simulink model "FOCwithLOAD"  (R2024b)
settings: Solver=FixedStepDiscrete  StartTime=0.0  StopTime=inf  RelTol=1e-3
PreLoadFcn:
  | % 自动加载同目录下的 linear_data.m，确保换机/首次打开可直接更新与编译
  | if ~evalin('base', 'exist(''Ts'',''var'') && exist(''pmsm'',''var'') && exist(''SMRC_I_Vsat_thresh'',''var'')')
  |     mdlDir_ = '';
  |     if bdIsLoaded('FOCwithLOAD'), mdlDir_ = fileparts(get_param('FOCwithLOAD', 'FileName')); end
  |     if isempty(mdlDir_), mdlDir_ = fileparts(which('FOCwithLOAD')); end
  |     if isempty(mdlDir_), mdlDir_ = pwd; end
  |     dataFile_ = fullfile(mdlDir_, 'linear_data.m');
  |     if isfile(dataFile_)
  |         assignin('base', 'linearDataFileTmp_', dataFile_);
  |         evalin('base', 'run(linearDataFileTmp_); clear linearDataFileTmp_');
  |     end
  |     clear mdlDir_ dataFile_
  | end
InitFcn:
  | % 自动加载同目录下的 linear_data.m，确保换机/首次打开可直接更新与编译
  | if ~evalin('base', 'exist(''Ts'',''var'') && exist(''pmsm'',''var'') && exist(''SMRC_I_Vsat_thresh'',''var'')')
  |     mdlDir_ = '';
  |     if bdIsLoaded('FOCwithLOAD'), mdlDir_ = fileparts(get_param('FOCwithLOAD', 'FileName')); end
  |     if isempty(mdlDir_), mdlDir_ = fileparts(which('FOCwithLOAD')); end
  |     if isempty(mdlDir_), mdlDir_ = pwd; end
  |     dataFile_ = fullfile(mdlDir_, 'linear_data.m');
  |     if isfile(dataFile_)
  |         assignin('base', 'linearDataFileTmp_', dataFile_);
  |         evalin('base', 'run(linearDataFileTmp_); clear linearDataFileTmp_');
  |     end
  |     clear mdlDir_ dataFile_
  | end
values from neighbouring files (symbols this model uses):
  a_hat = Kt_eff / (pmsm.J * omega_pu_base)    [linear_data.m]
  ADRC_B0 = 6055    [linear_data.m]
  ADRC_Wc = 3.2e-3    (= 0.0032)    [linear_data.m]
  ADRC_Wo = 30    [linear_data.m]
  alpha_ppc = exp(-lambda_ppc*Ts_speed)    [linear_data.m]
  b_hat = pmsm.B/pmsm.J    [linear_data.m]
  beta1 = single(2.0 * w_o)    [linear_data.m]
  beta2_sat_scale = 0.2    [linear_data.m]
  dataType = 'single'    [linear_data.m]
  gamma_reset = 0.9    [linear_data.m]
  inv_a_hat = 1/double(a_hat)    [linear_data.m]
  k_xi = 55    [linear_data.m]
  Kff = 0.98931745    [linear_data.m]
  lambda_ppc = 45    [linear_data.m]
  P_inf_const = 0.004    [linear_data.m]
  PI_params = mcb_SetControllerParameters(pmsm,inverter,PU_System,T_pwm,Ts,Ts_speed)    [linear_data.m]
  pmsm2 = pmsm    [linear_data.m]
  s_limit_sat = 0.9    [linear_data.m]
  speedRPM2mmps = pmlsm.mmps_per_rpm    [linear_data.m]
  target = mcb_SetProcessorDetails('F28379D',PWM_frequency)    [linear_data.m]
  Ts = T_pwm    (= 5e-05)    [linear_data.m]
  Ts_motor = T_pwm/2    (= 2.5e-05)    [linear_data.m]
  Ts_speed = 1*Ts    (= 5e-05)    [linear_data.m]
  w_o = single(200.0)    [linear_data.m]
  z2_limit = single(100.0)    [linear_data.m]
undefined symbols (not defined in the file or in its folder): DiscIntNeverNeededParam, Down, GPTRIP1SEL, GPTRIP2SEL, innerPI, inverter, inverter2, outerPI, pmlsm, pmsm, Tctr, TZ1, TZ2, Up
libraries: c2802xlib x13, simulink x10, c2837xDlib x6, c280xlib x6, slpidlib x5, svdschedulerlib x4, mcbcontrolslib x4, mcbpositiondecoderlib x2, mcbpmsmnonlinearlib x2, autolibpmsmexterior x2, mcbplantlib x2, svdutilitieslib x1
(part 2 of 5)

== system FOCwithLOAD/Motor2 Torque control/Control_System ==
  speed_RPM : Inport
  Iabc_meas_Real : Inport  Port=2
  Pos_PU : Inport  Port=3
  EnClosedLoop : Inport  Port=4
  Idq_ref_Real : Inport  Port=5
  AlignMode2Read : DataStoreRead  DataStoreName=AlignMode2  IndexOptions=Index vector (dialog)  Indices=1  OutputSizes=1
  AlignTheta2Read : DataStoreRead  DataStoreName=AlignTheta2  IndexOptions=Index vector (dialog)  Indices=1  OutputSizes=1
  Closed Loop Control1 : Subsystem  TreatAsAtomicUnit=on
  Switch : Switch  Criteria=u2 > Threshold  Threshold=0.5  SaturateOnIntegerOverflow=off  InputSameDT=off
  ThetaSw : Switch  Criteria=u2 > Threshold  Threshold=0.5  SaturateOnIntegerOverflow=off  InputSameDT=off
  ZeroOL : Constant  Value=0  OutDataTypeStr=single
  Duty_ABC : Outport  VectorParamsAs1DForOutWhenUnconnected=off
  VIdq_debug : Outport  Port=2  VectorParamsAs1DForOutWhenUnconnected=off
  wires:
  speed_RPM/1 -> Closed Loop Control1/3(Speed(RPM))
  AlignMode2Read/1 -> ThetaSw/2
  Pos_PU/1 -> ThetaSw/3
  Closed Loop Control1/2(VIdq_debug) -> VIdq_debug/1
  EnClosedLoop/1 -> Closed Loop Control1/Enable, Switch/2
  Idq_ref_Real/1 -> Closed Loop Control1/4(IdqRef)
  Iabc_meas_Real/1 -> Closed Loop Control1/1(Iabc)
  ThetaSw/1 -> Closed Loop Control1/2(Thetae_Sensor(0-1))
  Closed Loop Control1/1(Duty) -> Switch/1
  ZeroOL/1 -> Switch/3
  Switch/1 -> Duty_ABC/1
  AlignTheta2Read/1 -> ThetaSw/1

== system FOCwithLOAD/Motor2 Torque control/HW_Inputs ==
  Sim : Inport
  Sensor Driver Blocks (codegen) : Subsystem  VariantControl=(codegen)
  Sensor Driver Blocks (sim) : Subsystem  VariantControl=(sim)
  Out : Outport

== system FOCwithLOAD/Motor2 Torque control/Input Scaling ==
  note: Current Measurements
  note: Position & Speed Measurements
  note: QEP
  Ia_ADC : Inport
  Ib_ADC : Inport  Port=2
  Ic_ADC : Inport  Port=3
  QEP_Position_Count : Inport  Port=4
  QEP_Index_Latch : Inport  Port=5
  " Calculate Position and Speed" : Subsystem
  Calculate Phase Currents : Subsystem
  UnusedOffset : Constant  Value=0
  speed_RPM : Outport
  Iabc_meas_Real : Outport  Port=2
  Pos_PU : Outport  Port=3
  Motor2IndexFound : Outport  Port=4
  wires:
  Calculate Phase Currents/1(Iabc_meas_Real) -> Iabc_meas_Real/1  "Iabc_fb_Real"
  Ia_ADC/1 -> Calculate Phase Currents/1(Ia_ADC)
  Ib_ADC/1 -> Calculate Phase Currents/2(Ib_ADC)
  Ic_ADC/1 -> Calculate Phase Currents/3(Ic_ADC)
  QEP_Position_Count/1 -> " Calculate Position and Speed"/1(QEP_Position_Count)
  QEP_Index_Latch/1 -> " Calculate Position and Speed"/2(QEP_Index_Latch)
  UnusedOffset/1 -> " Calculate Position and Speed"/3(Offset)
  " Calculate Position and Speed"/1(Theta_e) -> Pos_PU/1
  " Calculate Position and Speed"/2(speed) -> speed_RPM/1
  " Calculate Position and Speed"/3(IndexFound) -> Motor2IndexFound/1

== system FOCwithLOAD/Motor2 Torque control/Inverter ==
  Inverter Signals : Inport
  Code Generation : Subsystem  VariantControl=(codegen)
  Simulation : Subsystem  VariantControl=(sim)
  DutyCycles : Outport  VectorParamsAs1DForOutWhenUnconnected=off

== system FOCwithLOAD/Motor2 Torque control/Output Scaling ==
  DutyABC : Inport
  Data Store Read : DataStoreRead  DataStoreName=EnMtr2Ctrl  IndexOptions=Index vector (dialog)  Indices=1  OutputSizes=1
  Data Type Conversion : DataTypeConversion  OutDataTypeStr=dataType  SaturateOnIntegerOverflow=off  RndMeth=Floor
  PWM_Duty_Cycles : Outport
  PWM_Enable : Outport  Port=2
  wires:
  Data Store Read/1 -> Data Type Conversion/1  "PWM_En"
  Data Type Conversion/1 -> PWM_Enable/1
  DutyABC/1 -> PWM_Duty_Cycles/1

== system FOCwithLOAD/Motor2 Torque control/align ==
  Iq_ref_real : Inport
  AlignMode2Read : DataStoreRead  DataStoreName=AlignMode2  IndexOptions=Index vector (dialog)  Indices=1  OutputSizes=1
  Constant : Constant  Value=0  OutDataTypeStr=single
  IdAlign2 : Constant  Value=1.5  OutDataTypeStr=single
  IdSw2 : Switch  Threshold=0.5  SaturateOnIntegerOverflow=off  InputSameDT=off
  IqSw2 : Switch  Threshold=0.5  SaturateOnIntegerOverflow=off  InputSameDT=off
  Mux1 : Mux  Inputs=2
  Out1 : Outport
  wires:
  Mux1/1 -> Out1/1
  IqSw2/1 -> Mux1/2
  IdSw2/1 -> Mux1/1
  Constant/1 -> IqSw2/1, IdSw2/3
  IdAlign2/1 -> IdSw2/1
  AlignMode2Read/1 -> IdSw2/2, IqSw2/2
  Iq_ref_real/1 -> IqSw2/3

== system FOCwithLOAD/Serial Receive/Parse SCI Rx ==
  Rx : Inport
  CalModeDTC : DataTypeConversion  OutDataTypeStr=uint8  RndMeth=Floor
  CalModeWrite : DataStoreWrite  DataStoreName=CalMode  IndexOptions=Index vector (dialog)  Indices=1  OutputSizes=1
  Data Store Memory : DataStoreMemory  DataStoreName=Enable_Real  WriteAfterWriteMsg=warning  ShowAdditionalParam=off
  Data Store Write : DataStoreWrite  DataStoreName=Enable  IndexOptions=Index vector (dialog)  Indices=1  OutputSizes=1
  Data Store Write1 : DataStoreWrite  DataStoreName=SpeedRef  IndexOptions=Index vector (dialog)  Indices=1  OutputSizes=1
  Data Store Write2 : DataStoreWrite  DataStoreName=Debug_signals  IndexOptions=Index vector (dialog)  Indices=1  OutputSizes=1
  Data_Conditioning_Rx : Subsystem  Variant=on
  ModeSrc : DataTypeConversion  OutDataTypeStr=uint16
  ModeWrite1 : DataStoreWrite  DataStoreName=Mode  IndexOptions=Index vector (dialog)  Indices=1  OutputSizes=1
  unParse : Subsystem
  Desired Speed : Outport  VectorParamsAs1DForOutWhenUnconnected=off
  Desried Iq ref : Outport  Port=2  VectorParamsAs1DForOutWhenUnconnected=off
  wires:
  unParse/1(Enable_PWM) -> Data Store Write/1, ModeSrc/1
  Data_Conditioning_Rx/1(Desired Speed) -> Desired Speed/1, Data Store Write1/1
  Data_Conditioning_Rx/3(Desired torque) -> Desried Iq ref/1
  unParse/2(Debug_signals) -> Data Store Write2/1
  Data_Conditioning_Rx/2(Out2) -> unParse/1(Data)
  Rx/1 -> Data_Conditioning_Rx/1(Rx)
  ModeSrc/1 -> ModeWrite1/1
  unParse/3(CalMode) -> CalModeDTC/1
  CalModeDTC/1 -> CalModeWrite/1

== system FOCwithLOAD/Serial Receive/Serial Receive ==
  Serial Rx : Subsystem  Variant=on
  Rx : Outport
  wires:
  Serial Rx/1(Rx) -> Rx/1

== system FOCwithLOAD/Serial Receive/Signal Packing ==
  note: 仿真侧复现上位机的 0/1 命令序列：
      |  t<0.5s  Enable_PWM=1 -> AlignFSM 对齐(锁存 PosOffset)
      |  t>=0.5s Enable_PWM=0 -> EnClosedLoop=1 闭环 PI
      | 恒为 1 时电机永远停在对齐态(Id=0.5PU, 速度≈0)
  Speedref : Inport
  IqRef : Inport  Port=2
  CalCmdSum : Sum
  Data_Conditioning_Tx : Subsystem  Variant=on
  Debug_signals : Constant  OutDataTypeStr=uint16  SampleTime=-1
  EnableCmd : Step  Time=1.3  Before=1  After=2
  EnableCmd2 : Step  Time=2.6  After=-2
  EnableCmdU16 : DataTypeConversion  OutDataTypeStr=uint16  SaturateOnIntegerOverflow=off  RndMeth=Floor
  Gain : Gain  Gain=1/pmsm.N_max
  Parse : Subsystem
  Data : Outport
  wires:
  Parse/1(Data) -> Data_Conditioning_Tx/2(In2)
  Debug_signals/1 -> Parse/2(Debug_signals)
  Speedref/1 -> Gain/1
  Data_Conditioning_Tx/1(Data) -> Data/1
  IqRef/1 -> Data_Conditioning_Tx/3(IqRef)
  Gain/1 -> Data_Conditioning_Tx/1(Speedref)
  EnableCmdU16/1 -> Parse/1(Enable_PWM)
  CalCmdSum/1 -> EnableCmdU16/1
  EnableCmd2/1 -> CalCmdSum/2
  EnableCmd/1 -> CalCmdSum/1

== system FOCwithLOAD/Simulation/Simulation1 ==
  Trigger : TriggerPort  VariantControl=Variant  PortDimensions=1
  ADCINT1 : simulink/Ports & Subsystems/Function-Call Generator  sample_time=-1  numberOfIterations=1  DisallowWideOutput=off
  Interrupt : Outport
  wires:
  ADCINT1/1 -> Interrupt/1

== system FOCwithLOAD/Simulation/Simulation2 ==
  Trigger : TriggerPort  VariantControl=Variant  PortDimensions=1
  ADCINT1 : simulink/Ports & Subsystems/Function-Call Generator  sample_time=-1  numberOfIterations=1  DisallowWideOutput=off
  Interrupt : Outport
  wires:
  ADCINT1/1 -> Interrupt/1

== system FOCwithLOAD/Hardware Init/Variant Subsystem/Code Generation ==
  note: for BoostXL-DRV8305 connected to LaunchXL-28379D
  note: System Outputs
  DRV Enable : Subsystem  Priority=1

== system FOCwithLOAD/Hardware Init/Variant Subsystem/Simulation ==

== system FOCwithLOAD/Heartbeat LED/Heartbeat LED/Code generation ==
  In1 : Inport
  Digital Output : c2837xDlib/Digital Output  GPIO_Number=GPIO32~GPIO39  GPIO_Bit0=off  GPIO_BIT0_Toggle=on  GPIO_Bit1=off  GPIO_BIT1_Toggle=off  GPIO_Bit2=on  GPIO_BIT2_Toggle=on  GPIO_Bit3=off  GPIO_BIT3_Toggle=off  GPIO_Bit4=off  GPIO_BIT4_Toggle=off  GPIO_Bit5=off  GPIO_BIT5_Toggle=off  GPIO_Bit6=off  GPIO_BIT6_Toggle=off  GPIO_Bit7=off  GPIO_BIT7_Toggle=off
  wires:
  In1/1 -> Digital Output/1

== system FOCwithLOAD/Heartbeat LED/Heartbeat LED/Simulation ==
  In1 : Inport
  Simulation_Terminator : Terminator
  wires:
  In1/1 -> Simulation_Terminator/1

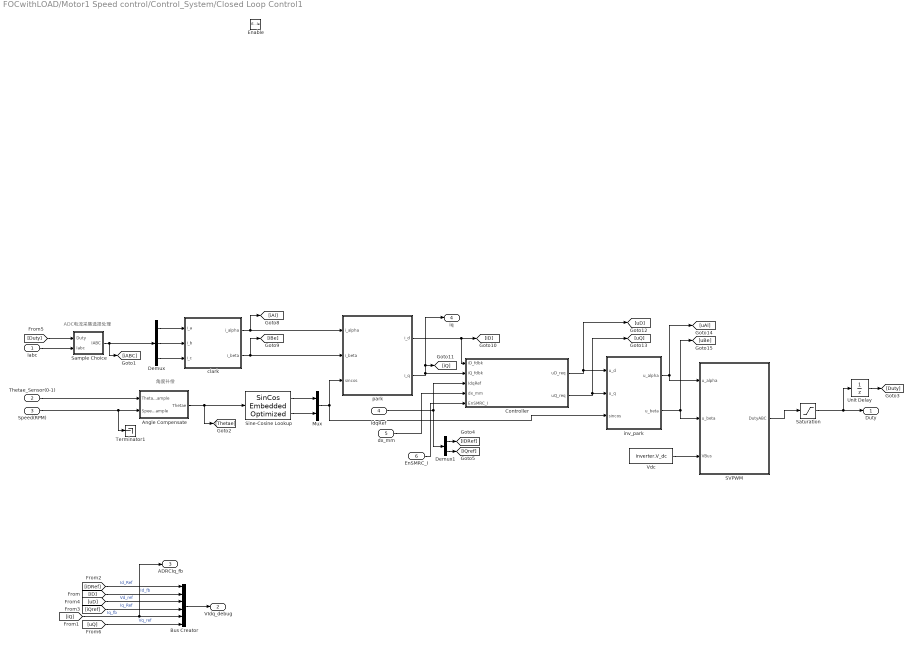
== system FOCwithLOAD/Motor1 Speed control/Control_System/Closed Loop Control1 ==
  note: 角度补偿
  note: ADC电流采集选择处理
  Iabc : Inport
  Thetae_Sensor(0-1) : Inport  Port=2
  Speed(RPM) : Inport  Port=3
  IdqRef : Inport  Port=4
  dx_mm : Inport  Port=5
  EnSMRC_I : Inport  Port=6
  Enable : EnablePort
  Angle Compensate : Subsystem
  Bus Creator : BusCreator  Inputs=6
  Controller : Subsystem
  Demux : Demux  Outputs=3
  Demux1 : Demux  Outputs=2
  Mux : Mux  Inputs=2
  SVPWM : Subsystem
      mask Display:
      | port_label('input',1,'u_{\alpha}','texmode','on');
      | port_label('input',2,'u_{\beta}','texmode','on');
      | port_label('input',3,'V_{Bus}','texmode','on');
      | 
      | port_label('output',1,'Duty_{ABC}','texmode','on');
      | 
      | fprintf('SVPWM');
  Sample Choice : Subsystem
  Saturation : Saturate  UpperLimit=1  LowerLimit=0
  Sine-Cosine Lookup : mcbcontrolslib/SinCos Embedded Optimized  LabelModeActiveChoice=MCB_Sin  OptforProc=off  ApproximationMethod=None  UserApproxMethod=Lookup  ApproxStatus=None  InterpMethod=Linear point-slope  NumberOfDataPoints=16  NumberOfIterations=11  RemoveProtectionAgainstOutOfRangeInput=off  TableDataTypeStr=Inherit: Inherit via input  AngleInput=Per-unit  ThetaDataType=single  N_points=1024  DatatypeInput=Inherit from input  Datatype=Inherit: Same as input
  Terminator1 : Terminator
  Unit Delay : UnitDelay  SampleTime=-1  HasFrameUpgradeWarning=on
  Vdc : Constant  Value=inverter.V_dc  OutDataTypeStr=single
  clark : Subsystem  TreatAsAtomicUnit=on
      mask Display:
      | port_label('input',1,'a','texmode','on');
      | port_label('input',2,'b','texmode','on');
      | port_label('input',3,'c','texmode','on');
      | 
      | port_label('output',1,'\alpha','texmode','on');
      | port_label('output',2,'\beta','texmode','on');
      | 
      | fprintf('Clark');
  inv_park : Subsystem
      mask Display:
      | port_label('input', 1, 'd', 'texmode', 'on');
      | port_label('input', 2, 'q', 'texmode', 'on');
      | port_label('input', 3, 'sin\theta_e cos\theta_e', 'texmode', 'on');
      | port_label('output', 1, '\alpha', 'texmode', 'on');
      | port_label('output', 2, '\beta', 'texmode', 'on');
      | fprintf('Inverse Park')
  park : Subsystem  TreatAsAtomicUnit=on
      mask Display:
      | port_label('input',1,'\alpha','texmode','on');
      | port_label('input',2,'\beta','texmode','on');
      | port_label('input',3,'sin\theta_e cos\theta_e','texmode','on');
      | 
      | port_label('output',1,'d','texmode','on');
      | port_label('output',2,'q','texmode','on');
      | 
      | fprintf('Park');
  Duty : Outport
  VIdq_debug : Outport  Port=2  VectorParamsAs1DForOutWhenUnconnected=off
  ADRCIq_fb : Outport  Port=3
  iq : Outport  Port=4  OutputWhenDisabled=reset  InitialOutput=0
  wires:
  inv_park/2(u_beta) -> [uBe], SVPWM/2(u_beta)
  Saturation/1 -> Unit Delay/1, Duty/1
  Demux/2 -> clark/2(i_b)
  Demux/3 -> clark/3(i_c)
  Mux/1 -> inv_park/3(sincos), park/3(sincos)
  Controller/2(uQ_req) -> inv_park/2(u_q), [uQ]
  SVPWM/1(DutyABC) -> Saturation/1
  park/1(i_d) -> [iD], Controller/1(iD_fdbk)
  Controller/1(uD_req) -> inv_park/1(u_d), [uD]
  clark/1(i_alpha) -> [iAl], park/1(i_alpha)
  clark/2(i_beta) -> [iBe], park/2(i_beta)
  inv_park/1(u_alpha) -> [uAl], SVPWM/1(u_alpha)
  park/2(i_q) -> Controller/2(iQ_fdbk), iq/1, [iQ]
  Demux/1 -> clark/1(i_a)
  Sine-Cosine Lookup/1 -> Mux/1
  Sine-Cosine Lookup/2 -> Mux/2
  [Duty] -> Sample Choice/1(Duty)
  Unit Delay/1 -> [Duty]
  Vdc/1 -> SVPWM/3(VBus)
  Speed(RPM)/1 -> Terminator1/1, Angle Compensate/2(SpeedSample)
  Thetae_Sensor(0-1)/1 -> Angle Compensate/1(ThetaeSample)
  Angle Compensate/1(Thetae) -> [Thetae], Sine-Cosine Lookup/1
  Iabc/1 -> Sample Choice/2(Iabc)
  Sample Choice/1(IABC) -> Demux/1, [iABC]
  IdqRef/1 -> Controller/3(IdqRef), Demux1/1
  [iD] -> Bus Creator/2  "Id_fb"
  Bus Creator/1 -> VIdq_debug/1
  [iDRef] -> Bus Creator/1  "Id_Ref"
  [uQ] -> Bus Creator/6  "Vq_ref"
  [uD] -> Bus Creator/3  "Vd_ref"
  [iQ] -> ADRCIq_fb/1, Bus Creator/5  "Iq_fb"
  [iQref] -> Bus Creator/4  "Iq_Ref"
  Demux1/1 -> [iDRef]
  Demux1/2 -> [iQref]
  EnSMRC_I/1 -> Controller/5(EnSMRC_I)
  dx_mm/1 -> Controller/4(dx_mm)

== system FOCwithLOAD/Motor1 Speed control/HW_Inputs/Sensor Driver Blocks (codegen) ==
  Sim : Inport
  ADC_A_IN2 : c2802xlib/ADC  Priority=2  blkParamProc=C2000_Type4  ADCModule=A  samplingMode=Single sample mode  ADCResolution=12-bit (Single-ended input)  useSOC1=SOC0  useSOC2=SOC0_SOC1  SOCAcquisitionWindow=30  SOCTriggerSource=ePWM1_ADCSOCA  SOCInterruptTrigger=No ADCINT  Ts=-1  dType=uint16  postInterrupt=off  interruptSel=ADCINT1  ADCINTContinuous=on  endma=off  chdma=1  conv1=ADCINA0  conv2=ADCINA0 and ADCINB0  conv1_Type4=ADCIN2  conv2_Type4=ADCIN0 and ADCIN1
  ADC_A_IN2_u32 : DataTypeConversion  OutDataTypeStr=uint32  SaturateOnIntegerOverflow=off  RndMeth=Floor
  ADC_B_IN2 : c2802xlib/ADC  Priority=3  blkParamProc=C2000_Type4  ADCModule=B  samplingMode=Single sample mode  ADCResolution=12-bit (Single-ended input)  useSOC1=SOC0  useSOC2=SOC0_SOC1  SOCAcquisitionWindow=30  SOCTriggerSource=ePWM1_ADCSOCA  SOCInterruptTrigger=No ADCINT  Ts=-1  dType=uint16  postInterrupt=on  interruptSel=ADCINT1  ADCINTContinuous=on  endma=off  chdma=1  conv1=ADCINA0  conv2=ADCINA0 and ADCINB0  conv1_Type4=ADCIN2  conv2_Type4=ADCIN0 and ADCIN1
  ADC_B_IN2_u32 : DataTypeConversion  OutDataTypeStr=uint32  SaturateOnIntegerOverflow=off  RndMeth=Floor
  ADC_C_IN2 : c2802xlib/ADC  Priority=1  blkParamProc=C2000_Type4  ADCModule=C  samplingMode=Single sample mode  ADCResolution=12-bit (Single-ended input)  useSOC1=SOC0  useSOC2=SOC0_SOC1  SOCAcquisitionWindow=30  SOCTriggerSource=ePWM1_ADCSOCA  SOCInterruptTrigger=No ADCINT  Ts=-1  dType=uint16  postInterrupt=off  interruptSel=ADCINT1  ADCINTContinuous=on  endma=off  chdma=1  conv1=ADCINA0  conv2=ADCINA0 and ADCINB0  conv1_Type4=ADCIN2  conv2_Type4=ADCIN0 and ADCIN1
  ADC_C_IN2_u32 : DataTypeConversion  OutDataTypeStr=uint32  SaturateOnIntegerOverflow=off  RndMeth=Floor
  Mux1 : Mux  Inputs=5
  Terminator : Terminator
  eQEP1 : c280xlib/eQEP  Priority=0  useModule=eQEP1  pcInputmode=Quadrature-count  externalClockrate=2x resolution: Count the rising/falling edge  swapPolarityselection=Clockwise  qdfOutputport=off  qapPolarityselection=off  qbpPolarityselection=off  qipPolarityselection=off  qspPolarityselection=off  igatePolarityselection=off  sampleTime=-1  pcOutputport=on  pcMaximumvalue=2^32-1  indexInitializationcheck=off  indexInitializationevent=Rising edge  strobeInitializationcheck=off  strobeInitializationevent=Rising edge  softwareInitializationcheck=off  softwareInitializationsource=Set to init value at start up  softwareInitializationmode=on  pcInitialvalue=0  pcResetmode=Reset on the maximum position  ieloutputport=on  indexEventlatch=Rising edge  seloutputport=off  strobeEventlatch=Rising edge  pcefOutputport=off  enableEqepcapture=off  qctmrOutputport=off  qcprdOutputport=off  captureTimerprescaler=128  upEventprescaler=128  overflowErrorflag=off  directionErrorflag=off  captureTimerposition=On position counter read  unitTimerperiod=100000000  captureTimerlatch=off  capturePeriodlatch=off  positionCounterlatch=off  soenPolarityselection=off  spselPolarityselection=Index pin is used for sync output  compareValuesource=Specify via dialog  shadowMode=Load on QPOSCNT=0  compareValue=4294967295  syncOutputwidth=1  polaritySyncoutput=Active high  watchdogEnable=off  watchdogTimer=65535  outport1Datatype=uint32  outport2Datatype=auto  outport3Datatype=auto  outport4Datatype=auto  outport5Datatype=auto  outport6Datatype=auto  outport7Datatype=auto  outport8Datatype=auto  outport9Datatype=auto  outport10Datatype=auto  outport11Datatype=auto  outport12Datatype=auto  eqepinterrupt_pce=off  eqepinterrupt_qpe=off  eqepinterrupt_qdc=off  eqepinterrupt_wto=off  eqepinterrupt_pcu=off  eqepinterrupt_pco=off  eqepinterrupt_pcr=off  eqepinterrupt_pcm=off  eqepinterrupt_sel=off  eqepinterrupt_iel=off  eqepinterrupt_uto=off  pheOutputport=off  watchdogOutputport=off  outport13Datatype=auto  outport14Datatype=auto
      settings: LibrarySourceBlock=c28002xlib/eQEP
  read_qep32 : CFunction  OutputCode=|  CodegenOutputCode=|
      OutputCode=|
      | /* 32-bit read: legacy c280xqep truncates QPOSCNT to uint16 */
      | y1 = (uint32_T)EQep1Regs.QPOSCNT;
      | y2 = (uint32_T)EQep1Regs.QPOSILAT;
      CodegenOutputCode=|
      | /* 32-bit read: legacy c280xqep truncates QPOSCNT to uint16 */
      | y1 = (uint32_T)EQep1Regs.QPOSCNT;
      | y2 = (uint32_T)EQep1Regs.QPOSILAT;
  term_eQEP1_1 : Terminator
  term_eQEP1_2 : Terminator
  Out : Outport
  wires:
  Mux1/1 -> Out/1
  Sim/1 -> Terminator/1
  ADC_A_IN2/1 -> ADC_A_IN2_u32/1
  ADC_A_IN2_u32/1 -> Mux1/1
  ADC_B_IN2/1 -> ADC_B_IN2_u32/1
  ADC_B_IN2_u32/1 -> Mux1/2
  ADC_C_IN2/1 -> ADC_C_IN2_u32/1
  ADC_C_IN2_u32/1 -> Mux1/3
  eQEP1/1 -> term_eQEP1_1/1
  eQEP1/2 -> term_eQEP1_2/1
  read_qep32/1 -> Mux1/4
  read_qep32/2 -> Mux1/5

== system FOCwithLOAD/Motor1 Speed control/HW_Inputs/Sensor Driver Blocks (sim) ==
  Sim : Inport
  Out : Outport
  wires:
  Sim/1 -> Out/1

== system FOCwithLOAD/Motor1 Speed control/Input Scaling/ Calculate Position and Speed ==
  note: 滤波
  note: 转速计算：(d*theta / dt)
  note: 计算出电角度
  QEP_Position_Count : Inport
  AlignFSM : MATLAB Function  TreatAsAtomicUnit=on
  AlignModeWrite : DataStoreWrite  DataStoreName=AlignMode  IndexOptions=Index vector (dialog)  Indices=1  OutputSizes=1
  AlignThetaWrite : DataStoreWrite  DataStoreName=AlignTheta  IndexOptions=Index vector (dialog)  Indices=1  OutputSizes=1
  EnClosedLoopWrite : DataStoreWrite  DataStoreName=EnClosedLoop  IndexOptions=Index vector (dialog)  Indices=1  OutputSizes=1
  EnableRead : DataStoreRead  DataStoreName=CalMode  IndexOptions=Index vector (dialog)  Indices=1  OutputSizes=1
  IIR Filter : mcbcontrolslib/IIR Filter  VariantControl=Low Pass Filter  VariantSelect=Low-pass  FilterConstantInputType=Specify via dialog  Filter_constant=0.1  advancedSettings=on  Ts=50e-6  cutOff_freq=353.6777
  ModPos : Math  Operator=mod
  One : Constant  OutDataTypeStr=single
  Pos2Ang : MATLAB Function  TreatAsAtomicUnit=on
  PosDelta : Subsystem
  PosOffsetWrite : DataStoreWrite  DataStoreName=PosOffset  IndexOptions=Index vector (dialog)  Indices=1  OutputSizes=1
  RunEnableRead : DataStoreRead  DataStoreName=Enable  IndexOptions=Index vector (dialog)  Indices=1  OutputSizes=1
  Speed Measurement : mcbpositiondecoderlib/Speed Measurement  PositionUnit=Per unit  PositionScalingDatatype=uint32  SpeedCalculationMode=Time interval for speed calculation  SampleTimeAsync=Ts  MaximumApplicationSpeed=6000  SpeedResolution=5e-6  DelayLength=20  MaximumMeasurableSpeed=29999  MeasurableSpeedResolution=1.397e-05  SpeedUnit=RPM  PerUnitSpeed=3000  SpeedDataType=dataType
  SumPos : Sum  Inputs=+-
  TsConst : Constant  Value=Ts  OutDataTypeStr=single
  Theta_e : Outport  VectorParamsAs1DForOutWhenUnconnected=off
  speed : Outport  Port=2  VectorParamsAs1DForOutWhenUnconnected=off
  QEP : Outport  Port=3
  theta_pu : Outport  Port=4
  dx_mm : Outport  Port=5
  wires:
  Speed Measurement/1 -> IIR Filter/1
  IIR Filter/1 -> speed/1
  SumPos/1 -> ModPos/1
  One/1 -> ModPos/2
  ModPos/1 -> Theta_e/1
  EnableRead/1 -> AlignFSM/1(Cmd)
  TsConst/1 -> AlignFSM/3(Ts)
  Pos2Ang/1(theta_pu) -> theta_pu/1, Speed Measurement/1, AlignFSM/2(PosRaw), SumPos/1, PosDelta/1(theta_pu)
  QEP_Position_Count/1 -> Pos2Ang/1(cnt), QEP/1
  AlignFSM/1(AlignMode) -> AlignModeWrite/1
  AlignFSM/2(EnClosedLoop) -> EnClosedLoopWrite/1
  PosDelta/1(dx_mm) -> dx_mm/1
  RunEnableRead/1 -> AlignFSM/4(EnRun)
  AlignFSM/4(AlignTheta) -> AlignThetaWrite/1
  AlignFSM/3(PosOffset) -> PosOffsetWrite/1, SumPos/2

== system FOCwithLOAD/Motor1 Speed control/Input Scaling/Calculate Phase Currents ==
  note: 增益放大
  note: 数模转换
  note: 校正
  note: 读取值
  note: 未启动时电流偏置
  Ia_ADC : Inport
  Ib_ADC : Inport  Port=2
  Ic_ADC : Inport  Port=3
  Add : Sum  Inputs=-+
  Data Store Read1 : DataStoreRead  DataStoreName=IaOffset_motor1  IndexOptions=Index vector (dialog)  Indices=1  OutputSizes=1
  Data Store Read2 : DataStoreRead  DataStoreName=IbOffset_motor1  IndexOptions=Index vector (dialog)  Indices=1  OutputSizes=1
  Data Store Read4 : DataStoreRead  DataStoreName=IcOffset_motor1  IndexOptions=Index vector (dialog)  Indices=1  OutputSizes=1
  Data Type Conversion : DataTypeConversion  OutDataTypeStr=int32  ConvertRealWorld=Stored Integer (SI)  RndMeth=Simplest  SaturateOnIntegerOverflow=off
  Data_Type : Subsystem  Variant=on
  Inverting / Non-inverting Current measurement amplifieer : Gain  Gain=inverter.invertingAmp  RndMeth=Simplest  OutDataTypeStr=Inherit: Same as input
  Mux : Mux  Inputs=3
  Mux1 : Mux  Inputs=3
  Iabc_meas_Real : Outport  VectorParamsAs1DForOutWhenUnconnected=off
  wires:
  Data Type Conversion/1 -> Add/2
  Data_Type/1(Iabc_meas_Real) -> Inverting / Non-inverting Current measurement amplifieer/1
  Ia_ADC/1 -> Mux/1
  Ib_ADC/1 -> Mux/2
  Mux/1 -> Data Type Conversion/1
  Data Store Read1/1 -> Mux1/1
  Data Store Read2/1 -> Mux1/2
  Mux1/1 -> Add/1
  Add/1 -> Data_Type/1(In1)
  Ic_ADC/1 -> Mux/3
  Data Store Read4/1 -> Mux1/3
  Inverting / Non-inverting Current measurement amplifieer/1 -> Iabc_meas_Real/1

== system FOCwithLOAD/Motor1 Speed control/Inverter/Code Generation ==
  note: for inverter connected with LaunchXL-28379D
  note: System Outputs
  Inverter Signals : Inport
  Constant : Constant  Value=inverter.EnableLogic
  DRV830x Enable : c2837xDlib/Digital Output  GPIO_Number=GPIO24~GPIO31  GPIO_Bit0=on  GPIO_BIT0_Toggle=off  GPIO_Bit1=off  GPIO_BIT1_Toggle=off  GPIO_Bit2=off  GPIO_BIT2_Toggle=off  GPIO_Bit3=off  GPIO_BIT3_Toggle=off  GPIO_Bit4=off  GPIO_BIT4_Toggle=off  GPIO_Bit5=off  GPIO_BIT5_Toggle=off  GPIO_Bit6=off  GPIO_BIT6_Toggle=off  GPIO_Bit7=off  GPIO_BIT7_Toggle=off
  Demux : Demux
  Demux1 : Demux  Outputs=3
  Ground : Ground
  Ground1 : Ground
  Ground2 : Ground
  Mux : Mux  Inputs=3
  Mux1 : Mux  Inputs=3
  Mux2 : Mux  Inputs=3
  NOT : Logic  Operator=NOT  IconShape=distinctive  AllPortsSameDT=off  OutDataTypeStr=boolean
  Scale_to_PWM_Counter_PRD : Gain  Gain=target.PWM_Counter_Period  OutDataTypeStr=uint16  RndMeth=Simplest
  Switch : Switch  Criteria=u2 > Threshold  SaturateOnIntegerOverflow=off  InputSameDT=off
  Switch1 : Switch  Threshold=0.5  SaturateOnIntegerOverflow=off  InputSameDT=off
  ePWM1 : c2802xlib/ePWM  PwmType=C2000_Type4  useModule=ePWM1  ePWMxLINKTBPRD=Not Linked  periodUnits=Clock cycles  timerSource=Specify via dialog  timerPeriod_clk=target.PWM_Counter_Period  timerPeriod_sec=0.0001  tbshadow=Counter equals to zero  countingMode=Up-Down  phaseActiveEnable=Disable  phaseDirection=Count down after sync  phaseActive=0  synchronizationEnable=off  dcaevt1Sync=off  dcbevt1Sync=off  synchronizationOption=Counter equals to zero (CTR=Zero)  dcbevt1SyncOut=off  dcaevt1SyncOut=off  cmpdSyncOut=off  cmpcSyncOut=off  cmpbSyncOut=off  zeroSyncOut=on  swfSyncOut=off  perSynchronizationOption=Counter equals to period (CTR=PRD)  clockPrescale=1  HSclockPrescale=1  enswap=off  ePWMxAStatus=on  ePWMxAactionLogic1=Do nothing  ePWMxAactionLogic2=Do nothing  ePWMxAactionLogic3=Clear  ePWMxAactionLogic4=Set  ePWMxAactionLogic5=Do nothing  ePWMxAactionLogic6=Do nothing  ePWMxACSFenable=off  ePWMxACSFvalue=Forcing disable  ePWMxASFreload=Zero  ePWMxBStatus=off  ePWMxBactionLogic1=Set  ePWMxBactionLogic2=Clear  ePWMxBactionLogic3=Do nothing  ePWMxBactionLogic4=Do nothing  ePWMxBactionLogic5=Clear  ePWMxBactionLogic6=Set  ePWMxBCSFenable=off  ePWMxBCSFvalue=Forcing disable  ePWMxBSFreload=Zero  ePWNxBOutWay=off  ePWMxLINKCMPA=Not Linked  CMPAUnits=Clock cycles  CMPASource=Input port  CMPAValue_per=50  CMPAValue_clk=floor(target.PWM_Counter_Period/2+1)  enCMPAshadow=Counter equals to zero (CTR=Zero)  ePWMxLINKCMPB=Not Linked  CMPBUnits=Clock cycles  CMPBSource=Specify via dialog  CMPBValue_per=50  CMPBValue_clk=floor(target.PWM_Counter_Period/2+1)  enCMPBshadow=Counter equals to zero (CTR=Zero)  ePWMxLINKCMPC=Not Linked  CMPCUnits=Clock cycles  CMPCSource=Specify via dialog  CMPCValue_per=50  CMPCValue_clk=32000  enCMPCshadow=Counter equals to zero (CTR=Zero)  ePWMxLINKCMPD=Not Linked  CMPDUnits=Clock cycles  CMPDSource=Specify via dialog  CMPDValue_per=50  CMPDValue_clk=32000  enCMPDshadow=Counter equals to zero (CTR=Zero)  enableDBePWMxA=on  enableDBePWMxB=on  enhalfcycle=off  DBpolarity=Active high complementary (AHC)  DBedgeDelay=Positive  DBSource_ePWMxA=ePWMxA  DBSource_ePWMxB=ePWMxA  DBPeriodUnits=Clock cycles  DBperiodSource=Input port  REDperiod=15  FEDperiod=15  REDperiod_sec=0  FEDperiod_sec=0  LoadModeDBRED=Immediate without using shadow  LoadModeDBFED=Immediate without using shadow  adcstartModuleA=on  adcrequestEventA=First event  adcstartEventA=Digital Compare Module A Event 1 start of conversion (DCAEVT1.soc)  adcstartEventA_type2=Counter equals to period (CTR=PRD)  adcstartModuleB=off  adcrequestEventB=First event  adcstartEventB=Counter equals to zero (CTR=Zero)  adcstartEventB_type2=Counter equals to zero (CTR=Zero)  intEn=off  intPrd=First event  intSel=Counter equals to zero (CTR=Zero)  intSel_type2=Counter equals to zero (CTR=Zero)  hrpe=off  enHRPWM=off  HRPWM_LoadMode=Counter equals to period (CTR=PRD)  HRPWM_CTLMode=Duty or Period control mode  HRPWM_EDGMode=Both edge  hrpeb=off  enHRPWMB=off  HRPWM_LoadModeB=Counter equals to zero (CTR=ZERO)  HRPWM_CTLModeB=Duty or Period control mode  HRPWM_EDGModeB=Both edge  enHRDBRED=off  enHRDBFED=off  enSFO=on  enautoconv=on  chopperEnable=off  chopperFrequency=1  chopperFirstwidth=1  chopperDuty=12.5%  tripZonesource=Specify via dialog  tzselOSHT1=off  tzselOSHT2=off  tzselOSHT3=off  tzselOSHT4=off  tzselOSHT5=off  tzselOSHT6=off  tzselOSHDCAEV1=off  tzselOSHDCBEV1=off  tzselCBC1=off  tzselCBC2=off  tzselCBC3=off  tzselCBC4=off  tzselCBC5=off  tzselCBC6=off  tzselCBCDCAEV2=off  tzselCBCDCBEV2=off  enTzOstIntr=off  enTzCbcIntr=off  enTzDCAEVT1Intr=off  enTzDCAEVT2Intr=off  enTzDCBEVT1Intr=off  enTzDCBEVT2Intr=off  tzclrCBCLatch=Counter equals to zero (CTR=Zero)  ePWMxAforced=No action  ePWMxBforced=No action  DCAEVT1forced=No action  DCBEVT1forced=No action  DCAEVT2forced=No action  DCBEVT2forced=No action  dcah=Trip Zone 1 input (TZ1)  dcal=Trip Zone 2 input (TZ2)  dcbh=Trip Zone 1 input (TZ1)  dcbl=Trip Zone 2 input (TZ2)  dcah_type2=GPTRIP1SEL/(TZ1)  dcal_type2=GPTRIP2SEL/(TZ2)  dcbh_type2=GPTRIP1SEL/(TZ1)  dcbl_type2=GPTRIP2SEL/(TZ2)  gendcaevt1=Event disabled  gendcaevt2=Event disabled  gendcbevt1=Event disabled  gendcbevt2=Event disabled  dcaevt1src=DCAEVT1 with sync  dcaevt2src=DCAEVT2 with sync  dcbevt1src=DCBEVT1 with sync  dcbevt2src=DCBEVT2 with sync  pulsesel=Counter equals to zero (CTR=Zero)  blankinv=off  blankoffset=0  blankwidth=0  evsrcsel=Filtered version of DCAEVT1 (DCAEVT1FILT)  encape=off
  ePWM2 : c2802xlib/ePWM  PwmType=C2000_Type4  useModule=ePWM2  ePWMxLINKTBPRD=Not Linked  periodUnits=Clock cycles  timerSource=Specify via dialog  timerPeriod_clk=target.PWM_Counter_Period  timerPeriod_sec=0.0001  tbshadow=Counter equals to zero  countingMode=Up-Down  phaseActiveEnable=Set counter to phase value specified via dialog  phaseDirection=Count up after sync  phaseActive=0  synchronizationEnable=off  dcaevt1Sync=off  dcbevt1Sync=off  synchronizationOption=Pass through (EPWMxSYNCI or SWFSYNC)  dcbevt1SyncOut=off  dcaevt1SyncOut=off  cmpdSyncOut=off  cmpcSyncOut=off  cmpbSyncOut=off  zeroSyncOut=off  swfSyncOut=on  perSynchronizationOption=Counter equals to period (CTR=PRD)  clockPrescale=1  HSclockPrescale=1  enswap=off  ePWMxAStatus=on  ePWMxAactionLogic1=Do nothing  ePWMxAactionLogic2=Do nothing  ePWMxAactionLogic3=Clear  ePWMxAactionLogic4=Set  ePWMxAactionLogic5=Do nothing  ePWMxAactionLogic6=Do nothing  ePWMxACSFenable=off  ePWMxACSFvalue=Forcing disable  ePWMxASFreload=Zero  ePWMxBStatus=off  ePWMxBactionLogic1=Set  ePWMxBactionLogic2=Clear  ePWMxBactionLogic3=Do nothing  ePWMxBactionLogic4=Do nothing  ePWMxBactionLogic5=Clear  ePWMxBactionLogic6=Set  ePWMxBCSFenable=off  ePWMxBCSFvalue=Forcing disable  ePWMxBSFreload=Zero  ePWNxBOutWay=off  ePWMxLINKCMPA=Not Linked  CMPAUnits=Clock cycles  CMPASource=Input port  CMPAValue_per=50  CMPAValue_clk=floor(target.PWM_Counter_Period/2+1)  enCMPAshadow=Counter equals to zero (CTR=Zero)  ePWMxLINKCMPB=Not Linked  CMPBUnits=Clock cycles  CMPBSource=Specify via dialog  CMPBValue_per=50  CMPBValue_clk=floor(target.PWM_Counter_Period/2+1)  enCMPBshadow=Counter equals to zero (CTR=Zero)  ePWMxLINKCMPC=Not Linked  CMPCUnits=Clock cycles  CMPCSource=Specify via dialog  CMPCValue_per=50  CMPCValue_clk=32000  enCMPCshadow=Counter equals to zero (CTR=Zero)  ePWMxLINKCMPD=Not Linked  CMPDUnits=Clock cycles  CMPDSource=Specify via dialog  CMPDValue_per=50  CMPDValue_clk=32000  enCMPDshadow=Counter equals to zero (CTR=Zero)  enableDBePWMxA=on  enableDBePWMxB=on  enhalfcycle=off  DBpolarity=Active high complementary (AHC)  DBedgeDelay=Positive  DBSource_ePWMxA=ePWMxA  DBSource_ePWMxB=ePWMxA  DBPeriodUnits=Clock cycles  DBperiodSource=Input port  REDperiod=15  FEDperiod=15  REDperiod_sec=0  FEDperiod_sec=0  LoadModeDBRED=Immediate without using shadow  LoadModeDBFED=Immediate without using shadow  adcstartModuleA=off  adcrequestEventA=First event  adcstartEventA=Digital Compare Module A Event 1 start of conversion (DCAEVT1.soc)  adcstartEventA_type2=Counter equals to period (CTR=PRD)  adcstartModuleB=off  adcrequestEventB=First event  adcstartEventB=Counter equals to zero (CTR=Zero)  adcstartEventB_type2=Counter equals to zero (CTR=Zero)  intEn=off  intPrd=First event  intSel=Counter equals to zero (CTR=Zero)  intSel_type2=Counter equals to zero (CTR=Zero)  hrpe=off  enHRPWM=off  HRPWM_LoadMode=Counter equals to period (CTR=PRD)  HRPWM_CTLMode=Duty or Period control mode  HRPWM_EDGMode=Both edge  hrpeb=off  enHRPWMB=off  HRPWM_LoadModeB=Counter equals to zero (CTR=ZERO)  HRPWM_CTLModeB=Duty or Period control mode  HRPWM_EDGModeB=Both edge  enHRDBRED=off  enHRDBFED=off  enSFO=on  enautoconv=on  chopperEnable=off  chopperFrequency=1  chopperFirstwidth=1  chopperDuty=12.5%  tripZonesource=Specify via dialog  tzselOSHT1=off  tzselOSHT2=off  tzselOSHT3=off  tzselOSHT4=off  tzselOSHT5=off  tzselOSHT6=off  tzselOSHDCAEV1=off  tzselOSHDCBEV1=off  tzselCBC1=off  tzselCBC2=off  tzselCBC3=off  tzselCBC4=off  tzselCBC5=off  tzselCBC6=off  tzselCBCDCAEV2=off  tzselCBCDCBEV2=off  enTzOstIntr=off  enTzCbcIntr=off  enTzDCAEVT1Intr=off  enTzDCAEVT2Intr=off  enTzDCBEVT1Intr=off  enTzDCBEVT2Intr=off  tzclrCBCLatch=Counter equals to zero (CTR=Zero)  ePWMxAforced=No action  ePWMxBforced=No action  DCAEVT1forced=No action  DCBEVT1forced=No action  DCAEVT2forced=No action  DCBEVT2forced=No action  dcah=Trip Zone 1 input (TZ1)  dcal=Trip Zone 2 input (TZ2)  dcbh=Trip Zone 1 input (TZ1)  dcbl=Trip Zone 2 input (TZ2)  dcah_type2=GPTRIP1SEL/(TZ1)  dcal_type2=GPTRIP2SEL/(TZ2)  dcbh_type2=GPTRIP1SEL/(TZ1)  dcbl_type2=GPTRIP2SEL/(TZ2)  gendcaevt1=Event disabled  gendcaevt2=Event disabled  gendcbevt1=Event disabled  gendcbevt2=Event disabled  dcaevt1src=DCAEVT1 with sync  dcaevt2src=DCAEVT2 with sync  dcbevt1src=DCBEVT1 with sync  dcbevt2src=DCBEVT2 with sync  pulsesel=Counter equals to zero (CTR=Zero)  blankinv=off  blankoffset=0  blankwidth=0  evsrcsel=Filtered version of DCAEVT1 (DCAEVT1FILT)  encape=off
  ePWM3 : c2802xlib/ePWM  PwmType=C2000_Type4  useModule=ePWM3  ePWMxLINKTBPRD=Not Linked  periodUnits=Clock cycles  timerSource=Specify via dialog  timerPeriod_clk=target.PWM_Counter_Period  timerPeriod_sec=0.0001  tbshadow=Counter equals to zero  countingMode=Up-Down  phaseActiveEnable=Set counter to phase value specified via dialog  phaseDirection=Count up after sync  phaseActive=0  synchronizationEnable=off  dcaevt1Sync=off  dcbevt1Sync=off  synchronizationOption=Pass through (EPWMxSYNCI or SWFSYNC)  dcbevt1SyncOut=off  dcaevt1SyncOut=off  cmpdSyncOut=off  cmpcSyncOut=off  cmpbSyncOut=off  zeroSyncOut=off  swfSyncOut=on  perSynchronizationOption=Counter equals to period (CTR=PRD)  clockPrescale=1  HSclockPrescale=1  enswap=off  ePWMxAStatus=on  ePWMxAactionLogic1=Do nothing  ePWMxAactionLogic2=Do nothing  ePWMxAactionLogic3=Clear  ePWMxAactionLogic4=Set  ePWMxAactionLogic5=Do nothing  ePWMxAactionLogic6=Do nothing  ePWMxACSFenable=off  ePWMxACSFvalue=Forcing disable  ePWMxASFreload=Zero  ePWMxBStatus=off  ePWMxBactionLogic1=Set  ePWMxBactionLogic2=Clear  ePWMxBactionLogic3=Do nothing  ePWMxBactionLogic4=Do nothing  ePWMxBactionLogic5=Clear  ePWMxBactionLogic6=Set  ePWMxBCSFenable=off  ePWMxBCSFvalue=Forcing disable  ePWMxBSFreload=Zero  ePWNxBOutWay=off  ePWMxLINKCMPA=Not Linked  CMPAUnits=Clock cycles  CMPASource=Input port  CMPAValue_per=50  CMPAValue_clk=floor(target.PWM_Counter_Period/2+1)  enCMPAshadow=Counter equals to zero (CTR=Zero)  ePWMxLINKCMPB=Not Linked  CMPBUnits=Clock cycles  CMPBSource=Specify via dialog  CMPBValue_per=50  CMPBValue_clk=floor(target.PWM_Counter_Period/2+1)  enCMPBshadow=Counter equals to zero (CTR=Zero)  ePWMxLINKCMPC=Not Linked  CMPCUnits=Clock cycles  CMPCSource=Specify via dialog  CMPCValue_per=50  CMPCValue_clk=32000  enCMPCshadow=Counter equals to zero (CTR=Zero)  ePWMxLINKCMPD=Not Linked  CMPDUnits=Clock cycles  CMPDSource=Specify via dialog  CMPDValue_per=50  CMPDValue_clk=32000  enCMPDshadow=Counter equals to zero (CTR=Zero)  enableDBePWMxA=on  enableDBePWMxB=on  enhalfcycle=off  DBpolarity=Active high complementary (AHC)  DBedgeDelay=Positive  DBSource_ePWMxA=ePWMxA  DBSource_ePWMxB=ePWMxA  DBPeriodUnits=Clock cycles  DBperiodSource=Input port  REDperiod=15  FEDperiod=15  REDperiod_sec=0  FEDperiod_sec=0  LoadModeDBRED=Immediate without using shadow  LoadModeDBFED=Immediate without using shadow  adcstartModuleA=off  adcrequestEventA=First event  adcstartEventA=Digital Compare Module A Event 1 start of conversion (DCAEVT1.soc)  adcstartEventA_type2=Counter equals to period (CTR=PRD)  adcstartModuleB=off  adcrequestEventB=First event  adcstartEventB=Counter equals to zero (CTR=Zero)  adcstartEventB_type2=Counter equals to zero (CTR=Zero)  intEn=off  intPrd=First event  intSel=Counter equals to zero (CTR=Zero)  intSel_type2=Counter equals to zero (CTR=Zero)  hrpe=off  enHRPWM=off  HRPWM_LoadMode=Counter equals to period (CTR=PRD)  HRPWM_CTLMode=Duty or Period control mode  HRPWM_EDGMode=Both edge  hrpeb=off  enHRPWMB=off  HRPWM_LoadModeB=Counter equals to zero (CTR=ZERO)  HRPWM_CTLModeB=Duty or Period control mode  HRPWM_EDGModeB=Both edge  enHRDBRED=off  enHRDBFED=off  enSFO=on  enautoconv=on  chopperEnable=off  chopperFrequency=1  chopperFirstwidth=1  chopperDuty=12.5%  tripZonesource=Specify via dialog  tzselOSHT1=off  tzselOSHT2=off  tzselOSHT3=off  tzselOSHT4=off  tzselOSHT5=off  tzselOSHT6=off  tzselOSHDCAEV1=off  tzselOSHDCBEV1=off  tzselCBC1=off  tzselCBC2=off  tzselCBC3=off  tzselCBC4=off  tzselCBC5=off  tzselCBC6=off  tzselCBCDCAEV2=off  tzselCBCDCBEV2=off  enTzOstIntr=off  enTzCbcIntr=off  enTzDCAEVT1Intr=off  enTzDCAEVT2Intr=off  enTzDCBEVT1Intr=off  enTzDCBEVT2Intr=off  tzclrCBCLatch=Counter equals to zero (CTR=Zero)  ePWMxAforced=No action  ePWMxBforced=No action  DCAEVT1forced=No action  DCBEVT1forced=No action  DCAEVT2forced=No action  DCBEVT2forced=No action  dcah=Trip Zone 1 input (TZ1)  dcal=Trip Zone 2 input (TZ2)  dcbh=Trip Zone 1 input (TZ1)  dcbl=Trip Zone 2 input (TZ2)  dcah_type2=GPTRIP1SEL/(TZ1)  dcal_type2=GPTRIP2SEL/(TZ2)  dcbh_type2=GPTRIP1SEL/(TZ1)  dcbl_type2=GPTRIP2SEL/(TZ2)  gendcaevt1=Event disabled  gendcaevt2=Event disabled  gendcbevt1=Event disabled  gendcbevt2=Event disabled  dcaevt1src=DCAEVT1 with sync  dcaevt2src=DCAEVT2 with sync  dcbevt1src=DCBEVT1 with sync  dcbevt2src=DCBEVT2 with sync  pulsesel=Counter equals to zero (CTR=Zero)  blankinv=off  blankoffset=0  blankwidth=0  evsrcsel=Filtered version of DCAEVT1 (DCAEVT1FILT)  encape=off
  stop : Constant  Value=0  OutDataTypeStr=uint16
  死区时间 : Constant  Value=15  OutDataTypeStr=uint16
  DutyCycles : Outport  VectorParamsAs1DForOutWhenUnconnected=off
  wires:
  Demux1/3 -> ePWM3/1  "PWM_C"
  Scale_to_PWM_Counter_PRD/1 -> Switch1/1
  Mux2/1 -> Switch1/3
  stop/1 -> Mux2/3, Mux2/2, Mux2/1
  Demux/4 -> Switch1/2, NOT/1, Switch/1  "Active high logic for inverter enable"
  Inverter Signals/1 -> Demux/1
  Demux1/2 -> ePWM2/1  "PWM_B"
  Switch1/1 -> Demux1/1
  Demux1/1 -> ePWM1/1  "PWM_A"
  Mux/1 -> Scale_to_PWM_Counter_PRD/1  "PWM Duty Cycles"
  Ground/1 -> Mux1/1
  Ground1/1 -> Mux1/3
  Ground2/1 -> Mux1/2
  Mux1/1 -> DutyCycles/1
  Demux/1 -> Mux/1
  Demux/2 -> Mux/2
  Demux/3 -> Mux/3
  Constant/1 -> Switch/2
  NOT/1 -> Switch/3  "Active low logic for inverter enable"
  Switch/1 -> DRV830x Enable/1
  死区时间/1 -> ePWM1/2, ePWM1/3, ePWM2/2, ePWM3/3, ePWM3/2, ePWM2/3

== system FOCwithLOAD/Motor1 Speed control/Inverter/Simulation ==
  Inverter Signals : Inport
  Data Type Duplicate : DataTypeDuplicate
  Demux : Demux
  Mux : Mux  Inputs=3
  Mux2 : Mux  Inputs=3
  Switch1 : Switch  Threshold=0.5  RndMeth=Simplest  SaturateOnIntegerOverflow=off  InputSameDT=off
  stop : Constant  Value=0  OutDataTypeStr=Inherit: Inherit via back propagation
  DutyCycles : Outport  VectorParamsAs1DForOutWhenUnconnected=off
  wires:
  stop/1 -> Data Type Duplicate/2, Mux2/1, Mux2/3, Mux2/2
  Mux2/1 -> Switch1/3
  Switch1/1 -> DutyCycles/1
  Inverter Signals/1 -> Demux/1
  Demux/4 -> Switch1/2  "PWM Enable"
  Mux/1 -> Data Type Duplicate/1, Switch1/1  "PWM Duty Cycles"
  Demux/1 -> Mux/1
  Demux/2 -> Mux/2
  Demux/3 -> Mux/3

== system FOCwithLOAD/Motor1 Speed control/Outer Controller/Subsystem ==
  SpeedPU_req : Inport
  SpeedPU_fdbk : Inport  Port=2
  Constant2 : Constant  Value=outerPI.Spd.Discrete.Kp  OutDataTypeStr=single
  Constant3 : Constant  Value=outerPI.Spd.Discrete.KiTctr  OutDataTypeStr=single
  Constant6 : Constant  Value=0  OutDataTypeStr=single
  Discrete PI Controller with anti-windup & reset : slpidlib/PID Controller  Controller=PI  Form=Parallel  TimeDomain=Discrete-time  UseExternalTs=off  SampleTime=-1  IntegratorMethod=Forward Euler  FilterMethod=Forward Euler  ControllerParametersSource=external  P=1  I=1  UseKiTs=on  D=0  UseExternalDerivativeSource=off  N=100  UseFilter=on  TunerSelectOption=Transfer Function Based (PID Tuner App)  InitialConditionSource=external  InitialConditionForIntegrator=0  InitialConditionForFilter=0  DifferentiatorICPrevScaledInput=0  ExternalReset=none  TrackingMode=off  Kt=1  LimitOutput=on  SatLimitsSource=internal  UpperSaturationLimit=9  LowerSaturationLimit=-9  LinearizeAsGain=on  AntiWindupMode=clamping  Kb=1  LimitIntegrator=off  UpperIntegratorSaturationLimit=inf  LowerIntegratorSaturationLimit=-inf  RndMeth=Simplest  POutMin=[]  POutMax=[]  IOutMin=[]  IOutMax=[]  DOutMin=[]  DOutMax=[]  NOutMin=[]  NOutMax=[]  SumOutMin=[]  SumOutMax=[]  SaturationOutDataTypeStr=Inherit: Inherit via back propagation  SaturationOutMin=[]  SaturationOutMax=[]  PParamMin=[]  PParamMax=[]  IParamMin=[]  IParamMax=[]  DParamMin=[]  DParamMax=[]  NParamMin=[]  NParamMax=[]  KbParamMin=[]  KbParamMax=[]  KtParamMin=[]  KtParamMax=[]  KbOutMin=[]  KbOutMax=[]  KtOutMin=[]  KtOutMax=[]  IntegratorOutMin=[]  IntegratorOutMax=[]  FilterOutMin=[]  FilterOutMax=[]  SumI1OutMin=[]  SumI1OutMax=[]  SumI2OutMin=[]  SumI2OutMax=[]  SumI3OutMin=[]  SumI3OutMax=[]  SumI4OutMin=[]  SumI4OutMax=[]  SumDOutMin=[]  SumDOutMax=[]  DifferentiatorOutMin=[]  DifferentiatorOutMax=[]  FilterDiffOutCoefMin=[]  FilterDiffOutCoefMax=[]  ReciprocalOutMin=[]  ReciprocalOutMax=[]  SumDenOutMin=[]  SumDenOutMax=[]  SumNumOutMin=[]  SumNumOutMax=[]  DivideOutMin=[]  DivideOutMax=[]  UdiffTsProdOutMin=[]  UdiffTsProdOutMax=[]  NTsProdOutMin=[]  NTsProdOutMax=[]  UintegralTsProdOutMin=[]  UintegralTsProdOutMax=[]  UngainTsProdOutMin=[]  UngainTsProdOutMax=[]  ClampingZeroOutDataTypeStr=Inherit: Inherit via back propagation  ClampingZeroOutMin=[]  ClampingZeroOutMax=[]  FilterDenConstantOutDataTypeStr=Inherit: Inherit via back propagation  FilterDenConstantOutMin=[]  FilterDenConstantOutMax=[]  PCopyOutDataTypeStr=Inherit: Inherit via back propagation  PCopyOutMin=[]  PCopyOutMax=[]  NCopyOutDataTypeStr=Inherit: Inherit via back propagation  NCopyOutMin=[]  NCopyOutMax=[]  IntegratorContinuousStateAttributes=''  IntegratorStateMustResolveToSignalObject=off  IntegratorRTWStateStorageClass=Auto  FilterContinuousStateAttributes=''  FilterStateMustResolveToSignalObject=off  FilterRTWStateStorageClass=Auto  ParallelPVariant=ExternalParameters  IdealPVariant=Disabled  IVariant=ExternalParameters  DVariant=Disabled  IntegratorVariant=Discrete  SatVariant=Enabled  AWVariant=DiscClampingParallel  PCopyVariant=Disabled  TRVariant=Disabled  FdbkBlocksVariant=Forward  IdealPFdbkVariant=Disabled  SatFdbkVariant=Disabled  DerivativeFilterVariant=Disabled  NVariant=Disabled  NCopyVariant=Disabled_SignalSpec  FilterICVariant=Disabled  IntegratorICVariant=ExternalICs  ExternalResetVariant=Disabled  TRSumVariant=Passthrough  SumFdbkVariant=Disabled  SumVariant=Sum_PI  TsampFilterVariant=InternalTs  TsampNgainVariant=Passthrough  TsampIntegralVariant=Disabled_SignalSpec  ExternalSaturationOutDataTypeStr=Inherit: Same as second input  DerivativeSourceVariant=Disabled  PreIntVariant=InternalPreInt
      settings: LibrarySourceBlock=mcbcontrolslib/PI Controller
  Sum : Sum  Inputs=|+-
  y : Outport
  wires:
  Constant2/1 -> Discrete PI Controller with anti-windup & reset/2
  Constant6/1 -> Discrete PI Controller with anti-windup & reset/4
  Constant3/1 -> Discrete PI Controller with anti-windup & reset/3
  Discrete PI Controller with anti-windup & reset/1 -> y/1
  Sum/1 -> Discrete PI Controller with anti-windup & reset/1
  SpeedPU_fdbk/1 -> Sum/2
  SpeedPU_req/1 -> Sum/1

== system FOCwithLOAD/Motor1 Speed control/Outer Controller/Subsystem1 ==
  SpeedPU_req : Inport
  SpeedPU_fdbk : Inport  Port=2
  ADCIq_fb : Inport  Port=3
  ADRC : Subsystem
  Data Type Conversion : DataTypeConversion  OutDataTypeStr=single  SaturateOnIntegerOverflow=off  RndMeth=Floor
  Mux : Mux  Inputs=2
  Unit Delay1 : UnitDelay  SampleTime=-1  HasFrameUpgradeWarning=on
  Iq_ref : Outport
  ESO : Outport  Port=2
  wires:
  ADRC/3(Z2_OUT) -> Mux/2
  ADCIq_fb/1 -> Unit Delay1/1
  Data Type Conversion/1 -> ESO/1
  Mux/1 -> Data Type Conversion/1
  ADRC/2(Z1_OUT) -> Mux/1
  Unit Delay1/1 -> ADRC/3(iqsync)
  SpeedPU_fdbk/1 -> ADRC/1(fdbPU)
  ADRC/1(Iq_ref) -> Iq_ref/1
  SpeedPU_req/1 -> ADRC/2(refPU)

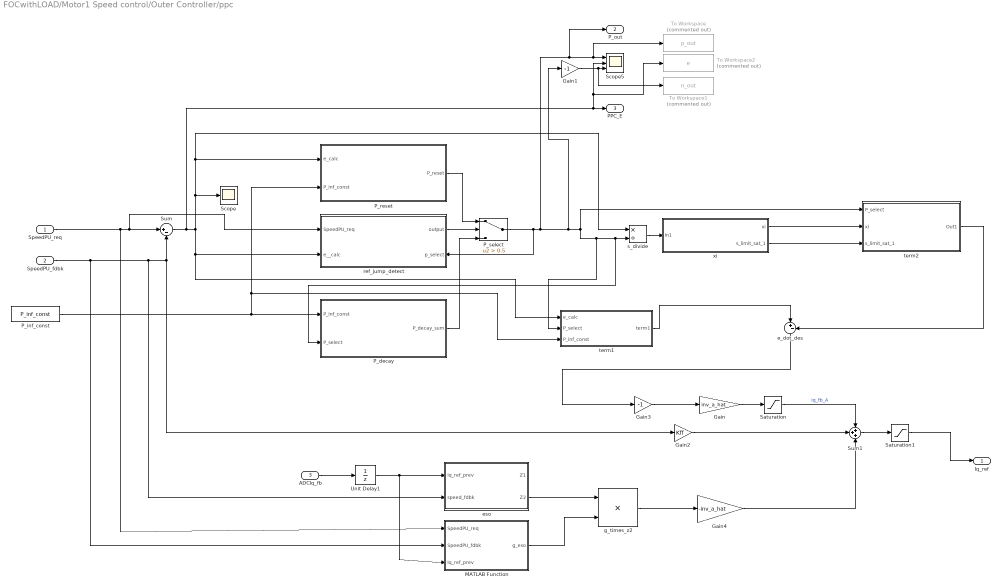
== system FOCwithLOAD/Motor1 Speed control/Outer Controller/ppc ==
  SpeedPU_req : Inport
  SpeedPU_fdbk : Inport  Port=2
  ADCIq_fb : Inport  Port=3
  Gain : Gain  Gain=inv_a_hat
  Gain1 : Gain  Gain=-1
  Gain2 : Gain  Gain=Kff
  Gain3 : Gain  Gain=-1
  Gain4 : Gain  Gain=-inv_a_hat  OutDataTypeStr=single
  MATLAB Function : MATLAB Function  TreatAsAtomicUnit=on
  P_decay : Subsystem
  P_inf_const : Constant  Value=P_inf_const
  P_reset : Subsystem
  P_select : Switch  Criteria=u2 > Threshold  Threshold=0.5  SaturateOnIntegerOverflow=off  InputSameDT=off
  Saturation : Saturate  UpperLimit=8  LowerLimit=-8  OutDataTypeStr=single
  Saturation1 : Saturate  UpperLimit=8  LowerLimit=-8
  Scope : Scope
  Scope5 : Scope  NumInputPorts=3
  Sum : Sum  Inputs=|+-
  Sum1 : Sum  Inputs=+++
  To Workspace : ToWorkspace  Commented=on  VariableName=p_out  SaveFormat=Timeseries  SampleTime=-1
  To Workspace1 : ToWorkspace  Commented=on  VariableName=n_out  SaveFormat=Timeseries  SampleTime=-1
  To Workspace2 : ToWorkspace  Commented=on  VariableName=e  SaveFormat=Timeseries  SampleTime=-1
  Unit Delay1 : UnitDelay  SampleTime=-1  HasFrameUpgradeWarning=on
  e_dot_des : Sum  Inputs=|+-
  eso : Subsystem
  g_times_z2 : Product
  ref_jump_detect : Subsystem
      settings: PortSchema="{\"entries\":[{\"content\":{\"sides\":[{\"content\":{\"connectorIds\":[\"In1\",\"In2\"]},\"type\":\"ConnectorPlacement.EquallySpacedRectSide\",\"uuid\":\"37563071-efd1-42ef-b9e0-d1a5b3b5012d\"},{\"content\":{\"connectorIds\":[\"Out1\",\"In3\"],\"side\":\"RIGHT\"},\"type\":\"ConnectorPlacement.EquallySpacedRectSide\",\"uuid\":\"bd9e4af0-e19c-46e0-b0aa-5a87a8fe2c09\"},{\"content\":{\"side\":\"TOP\"},\"type\":\"ConnectorPlacement.EquallySpacedRectSide\",\"uuid\":\"d41409f7-f51d-4a18-a4e6-1550d5e0894c\"}]},\"type\":\"ConnectorPlacement.EquallySpacedConnector\",\"uuid\":\"4c86894a-f3b6-4bd6-aa47-c4b058db0710\"}],\"packageUris\":[\"http://schema.mathworks.com/mf0/Connector/R2020b\"],\"version\":\"1.0\"}"
  s_divide : Product  Inputs=*/
  term1 : Subsystem
  term2 : Subsystem
  xi : Subsystem
  Iq_ref : Outport
  P_out : Outport  Port=2
  PPC_E : Outport  Port=3
  wires:
  SpeedPU_req/1 -> MATLAB Function/1(SpeedPU_req), ref_jump_detect/1(SpeedPU_req), Sum/1
  Sum/1 -> PPC_E/1, To Workspace2/1, Scope5/2, ref_jump_detect/2(e__calc), term1/1(e_calc), s_divide/1, P_reset/1(e_calc), Scope/1
  P_select/1 -> ref_jump_detect/3(p_select), Gain1/1, term1/2(P_select), P_decay/2(P_select), s_divide/2, term2/1(P_select), P_out/1, To Workspace/1, Scope5/1
  ref_jump_detect/1(output) -> P_select/2
  P_inf_const/1 -> P_reset/2(P_inf_const), term1/3(P_inf_const), P_decay/1(P_inf_const)
  P_reset/1(P_reset) -> P_select/1
  P_decay/1(P_decay_sum) -> P_select/3
  s_divide/1 -> xi/1(In1)
  xi/1(xi) -> term2/2(xi)
  SpeedPU_fdbk/1 -> MATLAB Function/2(SpeedPU_fdbk), Sum/2, Gain2/1, eso/2(speed_fdbk)
  e_dot_des/1 -> Gain3/1
  Gain/1 -> Saturation/1
  Saturation/1 -> Sum1/1  "iq_fb_A"
  term1/1(term1) -> e_dot_des/1
  term2/1(Out1) -> e_dot_des/2
  xi/2(s_limit_sat_1) -> term2/3(s_limit_sat_1)
  Gain1/1 -> To Workspace1/1, Scope5/3
  Gain3/1 -> Gain/1
  ADCIq_fb/1 -> Unit Delay1/1
  Unit Delay1/1 -> MATLAB Function/3(Iq_ref_prev), eso/1(Iq_ref_prev)
  eso/2(Z2) -> g_times_z2/1
  Gain2/1 -> Sum1/2
  Gain4/1 -> Sum1/3
  Sum1/1 -> Saturation1/1
  Saturation1/1 -> Iq_ref/1
  g_times_z2/1 -> Gain4/1
  MATLAB Function/1(g_eso) -> g_times_z2/2
